simulink model "FMS1"  (R2018b)
settings: configuration reference "fms_config" (kept outside this file)
values from neighbouring files (symbols this model uses):
  FMS_EXPORT = Simulink.Parameter(FMS_EXPORT_VALUE)    [fms_model_init.m]
  FMS_PARAM = Simulink.Parameter(FMS_PARAM_VALUE)    [fms_model_init.m]
undefined symbols (not defined in the file or in its folder): actuator_cmd, ax_cmd, ay_cmd, az_cmd, cmd_mask, ControlMode, ctrl_mode, DiscIntNeverNeededParam, FMS_Cmd, FMS_CONST, home, mode, p_cmd, phi_cmd, PilotMode, psi_rate_cmd, q_cmd, r_cmd, reset, state, status, theta_cmd, throttle_cmd, timestamp, u_cmd, v_cmd, VehicleState, VehicleStatus, w_cmd, wp_consume, wp_current
libraries: simulink x119, FMT_Model_Lib x56, hdlsllib x13
(part 1 of 7)
settings Model: Creator=jc  LastModifiedBy=zouji
settings ConfigSetRef: SourceLocation=Base Workspace

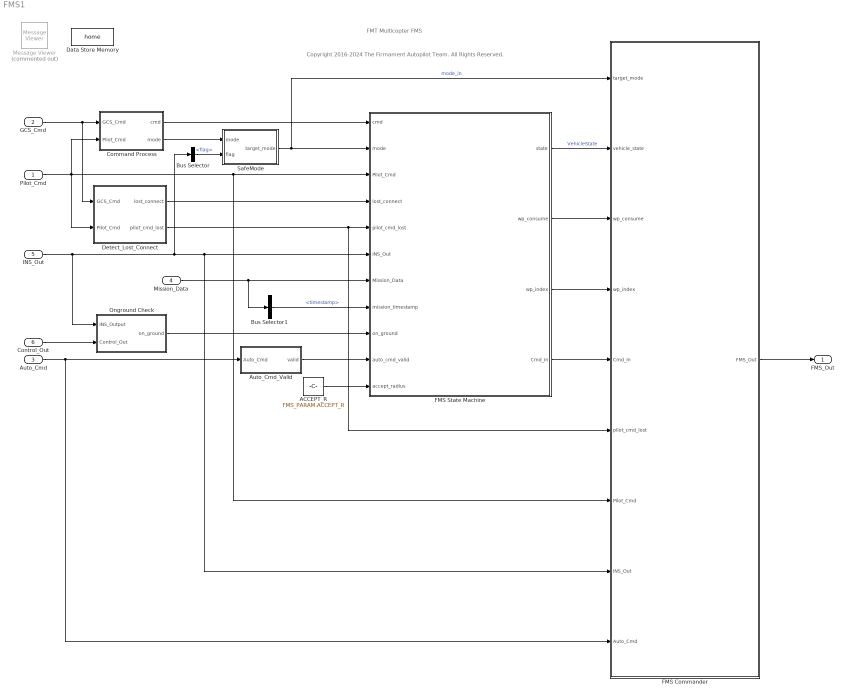
== system FMS1 ==
  note: Copyright 2016-2024 The Firmament Autopilot Team. All Rights Reserved.
  note: FMT Multicopter FMS
  Pilot_Cmd : Inport  OutDataTypeStr=Bus: Pilot_Cmd_Bus
  GCS_Cmd : Inport  Port=2  OutDataTypeStr=Bus: GCS_Cmd_Bus
  Auto_Cmd : Inport  Port=3  OutDataTypeStr=Bus: Auto_Cmd_Bus
  Mission_Data : Inport  Port=4  OutDataTypeStr=Bus: Mission_Data_Bus  BusOutputAsStruct=on
  INS_Out : Inport  Port=5  OutDataTypeStr=Bus: INS_Out_Bus
  Control_Out : Inport  Port=6  OutDataTypeStr=Bus: Control_Out_Bus
  ACCEPT_R : Constant  Value=FMS_PARAM.ACCEPT_R
  Auto_Cmd_Valid : Subsystem
  Bus Selector : BusSelector  OutputSignals=flag
  Bus Selector1 : BusSelector  OutputSignals=timestamp
  Command Process : Subsystem
  Data Store Memory : DataStoreMemory  DataStoreName=home  ReadBeforeWriteMsg=warning  WriteAfterWriteMsg=warning  WriteAfterReadMsg=warning  ShowAdditionalParam=off  OutDataTypeStr=single  Dimensions=4
  Detect_Lost_Connect : Subsystem
  FMS Commander : Subsystem  TreatAsAtomicUnit=on
  FMS State Machine : Stateflow chart  TreatAsAtomicUnit=on
  Message Viewer : MessageViewer  Commented=on  SavedRootId=#
  Onground Check : Subsystem
  SafeMode : Stateflow chart  TreatAsAtomicUnit=on
  FMS_Out : Outport  OutDataTypeStr=Bus: FMS_Out_Bus
  wires:
  Control_Out/1 -> Onground Check/2(Control_Out)
  Command Process/1(cmd) -> FMS State Machine/1(cmd)
  FMS State Machine/4(Cmd_In) -> FMS Commander/5(Cmd_In)
  Pilot_Cmd/1 -> Detect_Lost_Connect/2(Pilot_Cmd), FMS Commander/7(Pilot_Cmd), FMS State Machine/3(Pilot_Cmd), Command Process/2(Pilot_Cmd)
  INS_Out/1 -> Bus Selector/1, FMS Commander/8(INS_Out), FMS State Machine/6(INS_Out), Onground Check/1(INS_Output)
  Command Process/2(mode) -> SafeMode/1(mode)
  FMS Commander/1(FMS_Out) -> FMS_Out/1
  Onground Check/1(on_ground) -> FMS State Machine/9(on_ground)
  Bus Selector/1 -> SafeMode/2(flag)  "<flag>"
  GCS_Cmd/1 -> Command Process/1(GCS_Cmd), Detect_Lost_Connect/1(GCS_Cmd)
  SafeMode/1(target_mode) -> FMS Commander/1(target_mode), FMS State Machine/2(mode)  "mode_in"
  FMS State Machine/1(state) -> FMS Commander/2(vehicle_state)  "VehicleState"
  Mission_Data/1 -> Bus Selector1/1, FMS State Machine/7(Mission_Data)
  FMS State Machine/2(wp_consume) -> FMS Commander/3(wp_consume)
  Bus Selector1/1 -> FMS State Machine/8(mission_timestamp)  "<timestamp>"
  FMS State Machine/3(wp_index) -> FMS Commander/4(wp_index)
  ACCEPT_R/1 -> FMS State Machine/11(accept_radius)
  Auto_Cmd/1 -> FMS Commander/9(Auto_Cmd), Auto_Cmd_Valid/1(Auto_Cmd)
  Auto_Cmd_Valid/1(valid) -> FMS State Machine/10(auto_cmd_valid)
  Detect_Lost_Connect/1(lost_connect) -> FMS State Machine/4(lost_connect)
  Detect_Lost_Connect/2(pilot_cmd_lost) -> FMS Commander/6(pilot_cmd_lost), FMS State Machine/5(pilot_cmd_lost)

== system FMS1/Auto_Cmd_Valid ==
  Auto_Cmd : Inport
  Bus Selector1 : BusSelector  OutputSignals=frame
  Bus Selector2 : BusSelector  OutputSignals=timestamp
  Compare To Constant4 : simulink/Logic and Bit Operations/Compare To Constant  relop=<  const=1000  OutDataTypeStr=boolean
  Constant : Constant  Value=FMS_EXPORT.period  OutDataTypeStr=single
  Detect Change : simulink/Logic and Bit Operations/Detect Change  vinit=0  OutDataTypeStr=boolean
  Discrete-Time Integrator : DiscreteIntegrator  IntegratorMethod=Accumulation: Forward Euler  ExternalReset=sampled level  SampleTime=-1  OutDataTypeStr=uint32  SaturateOnIntegerOverflow=on  ICPrevOutput=DiscIntNeverNeededParam  ICPrevScaledInput=DiscIntNeverNeededParam
  Ever_Valid : Subsystem
  Interval Test : simulink/Logic and Bit Operations/Interval Test  IntervalClosedRight=on  uplimit=2  IntervalClosedLeft=on  lowlimit=0  OutDataTypeStr=boolean
  Logical Operator : Logic  Inputs=3  AllPortsSameDT=off  OutDataTypeStr=boolean
  valid : Outport
  wires:
  Constant/1 -> Discrete-Time Integrator/1
  Detect Change/1 -> Ever_Valid/1(in), Discrete-Time Integrator/2
  Discrete-Time Integrator/1 -> Compare To Constant4/1
  Auto_Cmd/1 -> Bus Selector1/1, Bus Selector2/1
  Compare To Constant4/1 -> Logical Operator/1
  Ever_Valid/1(out) -> Logical Operator/2
  Logical Operator/1 -> valid/1
  Bus Selector2/1 -> Detect Change/1  "<timestamp>"
  Bus Selector1/1 -> Interval Test/1  "<frame>"
  Interval Test/1 -> Logical Operator/3

== system FMS1/Command Process ==
  GCS_Cmd : Inport
  Pilot_Cmd : Inport  Port=2
  Check Valid : Subsystem
  Command PreProcess : Subsystem
  Mode PreProcess : Subsystem
  cmd : Outport
  mode : Outport  Port=2
  wires:
  GCS_Cmd/1 -> Mode PreProcess/2(GCS_Cmd), Command PreProcess/1(gcs_cmd)
  Pilot_Cmd/1 -> Command PreProcess/2(pilot_cmd), Check Valid/1(Pilot_Cmd), Mode PreProcess/3(Pilot_Cmd)
  Command PreProcess/1(cmd) -> cmd/1  "fms_cmd"
  Check Valid/1(pilot_cmd_valid) -> Mode PreProcess/1(pilot_cmd_valid)
  Mode PreProcess/1(mode) -> mode/1  "fms_mode"

== system FMS1/Detect_Lost_Connect ==
  GCS_Cmd : Inport
  Pilot_Cmd : Inport  Port=2
  Bus Selector : BusSelector  OutputSignals=timestamp
  Bus Selector1 : BusSelector  OutputSignals=timestamp
  Constant : Constant  Value=FMS_CONST.dt  OutDataTypeStr=single
  Constant1 : Constant  Value=FMS_PARAM.LOST_RETURN_EN
  Detect Change : simulink/Logic and Bit Operations/Detect Change  vinit=0  OutDataTypeStr=boolean
  Detect Change1 : simulink/Logic and Bit Operations/Detect Change  vinit=0  OutDataTypeStr=boolean
  Discrete-Time Integrator : DiscreteIntegrator  IntegratorMethod=Accumulation: Forward Euler  ExternalReset=sampled level  SampleTime=-1  OutDataTypeStr=single  SaturateOnIntegerOverflow=on  LimitOutput=on  UpperSaturationLimit=65535  LowerSaturationLimit=0  ICPrevOutput=DiscIntNeverNeededParam  ICPrevScaledInput=DiscIntNeverNeededParam
  Discrete-Time Integrator1 : DiscreteIntegrator  IntegratorMethod=Accumulation: Forward Euler  ExternalReset=sampled level  SampleTime=-1  OutDataTypeStr=single  SaturateOnIntegerOverflow=on  LimitOutput=on  UpperSaturationLimit=65535  LowerSaturationLimit=0  ICPrevOutput=DiscIntNeverNeededParam  ICPrevScaledInput=DiscIntNeverNeededParam
  Logical Operator : Logic  Operator=OR  Inputs=3  AllPortsSameDT=off  OutDataTypeStr=boolean
  Logical Operator1 : Logic  Operator=NOT  AllPortsSameDT=off  OutDataTypeStr=boolean
  Logical Operator2 : Logic  AllPortsSameDT=off  OutDataTypeStr=boolean
  timeout1_s : simulink/Logic and Bit Operations/Compare To Constant  relop=>=  const=FMS_PARAM.LOST_RETURN_TIME  OutDataTypeStr=boolean
  timeout2_s : simulink/Logic and Bit Operations/Compare To Constant  relop=>=  const=1  OutDataTypeStr=boolean
  lost_connect : Outport
  pilot_cmd_lost : Outport  Port=2
  wires:
  Constant/1 -> Discrete-Time Integrator1/1, Discrete-Time Integrator/1
  Discrete-Time Integrator/1 -> timeout1_s/1
  GCS_Cmd/1 -> Bus Selector/1
  Pilot_Cmd/1 -> Bus Selector1/1
  Bus Selector/1 -> Detect Change/1  "<timestamp>"
  Bus Selector1/1 -> Detect Change1/1  "<timestamp>"
  Detect Change/1 -> Logical Operator/1
  Detect Change1/1 -> Discrete-Time Integrator1/2, Logical Operator/2
  Constant1/1 -> Logical Operator2/2, Logical Operator1/1
  Logical Operator1/1 -> Logical Operator/3
  Logical Operator/1 -> Discrete-Time Integrator/2
  Logical Operator2/1 -> lost_connect/1
  timeout1_s/1 -> Logical Operator2/1
  Discrete-Time Integrator1/1 -> timeout2_s/1
  timeout2_s/1 -> pilot_cmd_lost/1

== system FMS1/FMS Commander ==
  target_mode : Inport
  vehicle_state : Inport  Port=2
  wp_consume : Inport  Port=3
  wp_index : Inport  Port=4
  Cmd_In : Inport  Port=5
  pilot_cmd_lost : Inport  Port=6
  Pilot_Cmd : Inport  Port=7
  INS_Out : Inport  Port=8
  Auto_Cmd : Inport  Port=9
  Commander : Subsystem
  FMS_Input : Subsystem  TreatAsAtomicUnit=on
  FMS_Out : Outport
  wires:
  target_mode/1 -> Commander/1(target_mode)
  FMS_Input/1(FMS_In) -> Commander/2(FMS_In)  "FMS_In"
  Commander/1(FMS_Out) -> FMS_Out/1
  vehicle_state/1 -> FMS_Input/1(state)
  wp_consume/1 -> FMS_Input/2(wp_consume)
  wp_index/1 -> FMS_Input/3(wp_index)
  Cmd_In/1 -> FMS_Input/4(Cmd_In)
  Pilot_Cmd/1 -> FMS_Input/6(Pilot_Cmd)
  INS_Out/1 -> FMS_Input/7(INS_Out)
  Auto_Cmd/1 -> FMS_Input/8(Auto_Cmd)
  pilot_cmd_lost/1 -> FMS_Input/5(pilot_cmd_lost)

== system FMS1/FMS State Machine/Vehicle.Arm.Auto.Mission.LLA2FLAT ==
  lla : Inport  OutDataTypeStr=double  PortDimensions=[1 3]
  llo : Inport  Port=2  OutDataTypeStr=double  Unit=deg  PortDimensions=[1 2]
  href : Inport  Port=3  OutDataTypeStr=double  Unit=m  PortDimensions=1
  psio : Inport  Port=4  OutDataTypeStr=double  Unit=deg  PortDimensions=1
  f : TriggerPort  TriggerType=function-call  VariantControl=(inherit)
      settings: CopyFcn=Stateflow.SLINSF.SimulinkMan.removeBlockPreDeleteFcn  PreDeleteFcn=Stateflow.SLINSF.SimulinkMan.unsafePredeleteFcn
  Data Type Conversion : DataTypeConversion  OutDataTypeStr=single
  LLA2FLAT : FMT_Model_Lib/Transformation/LLA2FLAT
      settings: SourceProductName=FMT Toolbox
  Signal Conversion : SignalConversion  OverrideOpt=off
  pos : Outport
  wires:
  LLA2FLAT/1 -> Signal Conversion/1
  lla/1 -> LLA2FLAT/1
  llo/1 -> LLA2FLAT/2
  href/1 -> LLA2FLAT/3
  psio/1 -> LLA2FLAT/4
  Signal Conversion/1 -> Data Type Conversion/1
  Data Type Conversion/1 -> pos/1

== system FMS1/FMS State Machine/Vehicle.PrepTakeoff ==
  xy_R : Inport  OutDataTypeStr=single  PortDimensions=2
  f : TriggerPort  TriggerType=function-call  VariantControl=(inherit)  StatesWhenEnabling=reset
      settings: CopyFcn=Stateflow.SLINSF.SimulinkMan.removeBlockPreDeleteFcn  PreDeleteFcn=Stateflow.SLINSF.SimulinkMan.unsafePredeleteFcn
  Constant : Constant  Value=FMS_PARAM.TAKEOFF_H
  Mux : Mux  Inputs=2
  Reshape : Reshape  OutputDimensionality=Column vector (2-D)
  sp_takeoff : Outport
  wires:
  Reshape/1 -> sp_takeoff/1
  xy_R/1 -> Mux/1
  Mux/1 -> Reshape/1
  Constant/1 -> Mux/2

== system FMS1/FMS State Machine/Vehicle.StickMoved ==
  stick_val : Inport  OutDataTypeStr=double  PortDimensions=4
  pilot_cmd : Inport  Port=2  OutDataTypeStr=Bus: Pilot_Cmd_Bus  PortDimensions=1
  f : TriggerPort  TriggerType=function-call  VariantControl=(inherit)
      settings: CopyFcn=Stateflow.SLINSF.SimulinkMan.removeBlockPreDeleteFcn  PreDeleteFcn=Stateflow.SLINSF.SimulinkMan.unsafePredeleteFcn
  Abs : Abs
  Bus Selector : BusSelector  OutputSignals=stick_yaw,stick_throttle,stick_roll,stick_pitch
  Compare To Constant : simulink/Logic and Bit Operations/Compare To Constant  relop=>=  const=0.1  OutDataTypeStr=boolean
  Max : MinMax  Function=max
  Mux : Mux
  Sum : Sum  Inputs=|+-
  moved : Outport
  wires:
  pilot_cmd/1 -> Bus Selector/1
  Bus Selector/1 -> Mux/1  "<stick_yaw>"
  Bus Selector/2 -> Mux/2  "<stick_throttle>"
  Bus Selector/3 -> Mux/3  "<stick_roll>"
  Bus Selector/4 -> Mux/4  "<stick_pitch>"
  stick_val/1 -> Sum/1
  Mux/1 -> Sum/2
  Sum/1 -> Abs/1
  Abs/1 -> Max/1
  Max/1 -> Compare To Constant/1
  Compare To Constant/1 -> moved/1

== system FMS1/Onground Check ==
  INS_Output : Inport
  Control_Out : Inport  Port=2
  Bus Selector : BusSelector  OutputSignals=quat
  Bus Selector1 : BusSelector  OutputSignals=actuator_cmd
  Bus Selector2 : BusSelector  OutputSignals=phi,theta
  Bus Selector3 : BusSelector  OutputSignals=ax,ay,az
  Constant : Constant  Value=4  OutDataTypeStr=uint16
  Cos : Trigonometry  Operator=cos
  Cos1 : Trigonometry  Operator=cos
  Divide : Product  Inputs=*/
  Divide1 : Product  Inputs=/*
  First Order LPF : FMT_Model_Lib/Filter/First Order LPF  fc=1/(2*pi*0.5)
      settings: SourceProductName=FMT Toolbox
  First Order LPF1 : FMT_Model_Lib/Filter/First Order LPF  fc=1/(2*pi*0.1)
      settings: SourceProductName=FMT Toolbox
  First Order LPF2 : FMT_Model_Lib/Filter/First Order LPF  fc=1/(2*pi*0.1)
      settings: SourceProductName=FMT Toolbox
  Interval Test : simulink/Logic and Bit Operations/Interval Test  IntervalClosedRight=on  uplimit=[0.5, 0.5, -9.806+0.5]  IntervalClosedLeft=on  lowlimit=[-0.5, -0.5, -9.806-0.5]  OutDataTypeStr=boolean
  Land_Lock_Thro : Constant  Value=FMS_PARAM.LAND_LOCK_THRO
  Logical Operator : Logic  Inputs=1  AllPortsSameDT=off  OutDataTypeStr=boolean
  Logical Operator1 : Logic  AllPortsSameDT=off  OutDataTypeStr=boolean
  Matrix Concatenate3 : Concatenate  NumInputs=3  ConcatenateDimension=2
  Multiply : Product  Multiplication=Matrix(*)
  Multiply1 : Product
  Quaternion To DCM : FMT_Model_Lib/Quaternion/Quaternion To DCM
      settings: SourceProductName=FMT Toolbox
  Relational Operator : RelationalOperator  Operator=<  OutDataTypeStr=boolean  RndMeth=Simplest
  Saturation : Saturate  UpperLimit=1  LowerLimit=0.9
  Selector : Selector  InputPortWidth=16  IndexOptions=Index vector (dialog)  Indices=[1:4]  OutputSizes=1
  Sum of Elements : Sum  Inputs=+
  Transpose : Math  Operator=transpose  SaturateOnIntegerOverflow=on
  on_ground : Outport
  wires:
  Bus Selector3/2 -> Matrix Concatenate3/2  "<ay>"
  Relational Operator/1 -> Logical Operator1/2
  Bus Selector3/3 -> Matrix Concatenate3/3  "<az>"
  Bus Selector1/1 -> Selector/1  "<actuator_cmd>"
  Bus Selector3/1 -> Matrix Concatenate3/1  "<ax>"
  Selector/1 -> Sum of Elements/1
  INS_Output/1 -> Bus Selector2/1, Bus Selector3/1, Bus Selector/1
  Control_Out/1 -> Bus Selector1/1
  Interval Test/1 -> Logical Operator/1
  Sum of Elements/1 -> Divide/1
  Constant/1 -> Divide/2
  First Order LPF/1 -> Interval Test/1
  Divide/1 -> First Order LPF2/1
  First Order LPF2/1 -> Relational Operator/1
  Logical Operator/1 -> Logical Operator1/1
  Logical Operator1/1 -> on_ground/1  "on_ground"
  Bus Selector/1 -> Quaternion To DCM/1  "<quat>"
  Quaternion To DCM/1 -> Transpose/1
  Matrix Concatenate3/1 -> Multiply/2
  Transpose/1 -> Multiply/1
  Multiply/1 -> First Order LPF/1
  Bus Selector2/1 -> Cos/1  "<phi>"
  Bus Selector2/2 -> Cos1/1  "<theta>"
  Cos/1 -> Multiply1/1
  Cos1/1 -> Multiply1/2
  Multiply1/1 -> Saturation/1
  Saturation/1 -> Divide1/1
  Divide1/1 -> First Order LPF1/1
  First Order LPF1/1 -> Relational Operator/2
  Land_Lock_Thro/1 -> Divide1/2

== system FMS1/Auto_Cmd_Valid/Ever_Valid ==
  in : Inport
  Constant1 : Constant  OutDataTypeStr=uint8
  Delay : Delay  DelayLength=1
  Switch : Switch  Criteria=u2 > Threshold
  out : Outport
  wires:
  Constant1/1 -> Switch/1
  Delay/1 -> Switch/3
  in/1 -> Switch/2
  Switch/1 -> out/1, Delay/1

== system FMS1/Command Process/Check Valid ==
  Pilot_Cmd : Inport
  Bus Selector1 : BusSelector  OutputSignals=timestamp
  Compare To Constant1 : simulink/Logic and Bit Operations/Compare To Constant  relop=<  const=500  OutDataTypeStr=boolean
  Constant1 : Constant  Value=FMS_EXPORT.period  OutDataTypeStr=single
  Detect Change1 : simulink/Logic and Bit Operations/Detect Change  vinit=0  OutDataTypeStr=boolean
  Discrete-Time Integrator1 : DiscreteIntegrator  IntegratorMethod=Accumulation: Forward Euler  ExternalReset=sampled level  SampleTime=-1  OutDataTypeStr=uint32  SaturateOnIntegerOverflow=on  ICPrevOutput=DiscIntNeverNeededParam  ICPrevScaledInput=DiscIntNeverNeededParam
  pilot_cmd_valid : Outport
  wires:
  Pilot_Cmd/1 -> Bus Selector1/1
  Compare To Constant1/1 -> pilot_cmd_valid/1
  Bus Selector1/1 -> Detect Change1/1  "<timestamp>"
  Constant1/1 -> Discrete-Time Integrator1/1
  Detect Change1/1 -> Discrete-Time Integrator1/2
  Discrete-Time Integrator1/1 -> Compare To Constant1/1

== system FMS1/Command Process/Command PreProcess ==
  gcs_cmd : Inport
  pilot_cmd : Inport  Port=2
  Bus Selector : BusSelector  OutputSignals=cmd_1
  Bus Selector1 : BusSelector  OutputSignals=cmd_1
  Bus Selector2 : BusSelector  OutputSignals=param
  Compare To Constant : simulink/Logic and Bit Operations/Compare To Constant  relop===  const=FMS_Cmd.SetHome  OutDataTypeStr=boolean
  Constant1 : Constant  Value=FMS_Cmd.None
  Data Type Conversion1 : DataTypeConversion  OutDataTypeStr=Enum: FMS_Cmd
  Data Type Conversion2 : DataTypeConversion  OutDataTypeStr=Enum: FMS_Cmd
  Detect Change3 : simulink/Logic and Bit Operations/Detect Change  vinit=0  OutDataTypeStr=boolean
  Detect Change4 : simulink/Logic and Bit Operations/Detect Change  vinit=0  OutDataTypeStr=boolean
  Selector : Selector  InputPortWidth=7  IndexOptions=Index vector (dialog)  Indices=[1:4]  OutputSizes=1
  SetHome : Subsystem  TreatAsAtomicUnit=on
  Switch1 : Switch  Criteria=u2 > Threshold
  Switch2 : Switch  Criteria=u2 > Threshold
  cmd : Outport
  wires:
  Bus Selector/1 -> Data Type Conversion1/1, Detect Change4/1  "<cmd_1>"
  pilot_cmd/1 -> Bus Selector1/1
  Switch1/1 -> cmd/1
  gcs_cmd/1 -> Bus Selector2/1, Bus Selector/1
  Bus Selector1/1 -> Data Type Conversion2/1, Detect Change3/1  "<cmd_1>"
  Detect Change3/1 -> Switch1/2
  Switch2/1 -> Switch1/3
  Detect Change4/1 -> Switch2/2
  Data Type Conversion2/1 -> Switch1/1
  Data Type Conversion1/1 -> Compare To Constant/1, Switch2/1
  Constant1/1 -> Switch2/3
  Compare To Constant/1 -> SetHome/Trigger
  Bus Selector2/1 -> Selector/1  "<param>"
  Selector/1 -> SetHome/1(home)

== system FMS1/Command Process/Mode PreProcess ==
  pilot_cmd_valid : Inport
  GCS_Cmd : Inport  Port=2
  Pilot_Cmd : Inport  Port=3
  Bus Selector1 : BusSelector  OutputSignals=mode
  Bus Selector2 : BusSelector  OutputSignals=mode
  Compare To Zero : simulink/Logic and Bit Operations/Compare To Zero  relop=~=  OutDataTypeStr=boolean
  Compare To Zero1 : simulink/Logic and Bit Operations/Compare To Zero  relop=~=  OutDataTypeStr=boolean
  Data Type Conversion1 : DataTypeConversion  OutDataTypeStr=Enum: PilotMode
  Data Type Conversion2 : DataTypeConversion  OutDataTypeStr=Enum: PilotMode
  Delay : Delay  DelayLength=1  InitialCondition=PilotMode.None
  Detect Change : simulink/Logic and Bit Operations/Detect Change  vinit=0  OutDataTypeStr=boolean
  Logical Operator : Logic  AllPortsSameDT=off  OutDataTypeStr=boolean
  Logical Operator1 : Logic  AllPortsSameDT=off  OutDataTypeStr=boolean
  Switch : Switch  Criteria=u2 > Threshold
  Switch1 : Switch  Criteria=u2 > Threshold
  mode : Outport
  wires:
  Bus Selector2/1 -> Compare To Zero/1, Detect Change/1, Data Type Conversion1/1  "<mode>"
  GCS_Cmd/1 -> Bus Selector2/1
  Pilot_Cmd/1 -> Bus Selector1/1
  Bus Selector1/1 -> Compare To Zero1/1, Data Type Conversion2/1  "<mode>"
  Logical Operator1/1 -> Switch/2
  Data Type Conversion2/1 -> Switch/1
  Switch/1 -> mode/1, Delay/1
  Delay/1 -> Switch1/3
  Compare To Zero/1 -> Logical Operator/2
  Data Type Conversion1/1 -> Switch1/1
  Switch1/1 -> Switch/3
  Detect Change/1 -> Logical Operator/1
  Logical Operator/1 -> Switch1/2
  pilot_cmd_valid/1 -> Logical Operator1/2
  Compare To Zero1/1 -> Logical Operator1/1

== system FMS1/FMS Commander/Commander ==
  target_mode : Inport
  FMS_In : Inport  Port=2
  Arm : Subsystem  TreatAsAtomicUnit=on
  Bus Selector1 : BusSelector  OutputSignals=vehicle_state
  Bus_Constructor : Subsystem
  Disarm : Subsystem  TreatAsAtomicUnit=on
  FMS_In1 : InportShadow  Port=2
  FMS_In2 : InportShadow  Port=2
  Merge : Merge  Inputs=3
  Standby : Subsystem  TreatAsAtomicUnit=on
  Switch Case : SwitchCase  CaseConditions={[VehicleState.Disarm,VehicleState.None], VehicleState.Standby}
  FMS_Out : Outport
  wires:
  Switch Case/3 -> Arm/Action
  Bus Selector1/1 -> Switch Case/1  "<vehicle_state>"
  FMS_In/1 -> Bus Selector1/1
  Standby/1(FMS_Out) -> Merge/2
  Arm/1(FMS_Out) -> Merge/3
  Switch Case/2 -> Standby/Action
  Switch Case/1 -> Disarm/Action
  Disarm/1(FMS_Out) -> Merge/1
  FMS_In1/1 -> Arm/1(FMS_In)
  Merge/1 -> Bus_Constructor/1(Bus_In)
  target_mode/1 -> Bus_Constructor/2(target_mode)
  FMS_In2/1 -> Bus_Constructor/3(FMS_In)
  Bus_Constructor/1(FMS_Out) -> FMS_Out/1

== system FMS1/FMS Commander/FMS_Input ==
  state : Inport
  wp_consume : Inport  Port=2
  wp_index : Inport  Port=3
  Cmd_In : Inport  Port=4
  pilot_cmd_lost : Inport  Port=5
  Pilot_Cmd : Inport  Port=6
  INS_Out : Inport  Port=7
  Auto_Cmd : Inport  Port=8
  Bus Creator : BusCreator  Inputs=8
  Signal Copy{,1..7} (8 alike) : SignalConversion  OverrideOpt=off
  FMS_In : Outport
  wires:
  Bus Creator/1 -> FMS_In/1
  Pilot_Cmd/1 -> Signal Copy2/1
  Auto_Cmd/1 -> Signal Copy/1
  INS_Out/1 -> Signal Copy1/1
  Signal Copy2/1 -> Bus Creator/6  "Pilot_Cmd"
  Signal Copy/1 -> Bus Creator/8  "Auto_Cmd"
  Signal Copy1/1 -> Bus Creator/7  "INS_Out"
  Cmd_In/1 -> Signal Copy3/1
  Signal Copy3/1 -> Bus Creator/4  "Cmd_In"
  wp_index/1 -> Signal Copy5/1
  Signal Copy5/1 -> Bus Creator/3  "wp_index"
  wp_consume/1 -> Signal Copy4/1
  Signal Copy4/1 -> Bus Creator/2  "wp_consume"
  state/1 -> Signal Copy6/1
  Signal Copy6/1 -> Bus Creator/1  "vehicle_state"
  pilot_cmd_lost/1 -> Signal Copy7/1
  Signal Copy7/1 -> Bus Creator/5  "pilot_cmd_lost"

== system FMS1/Command Process/Command PreProcess/SetHome ==
  home : Inport
  Trigger : TriggerPort  VariantControl=Variant
  Data Store Write : DataStoreWrite  DataStoreName=home
  wires:
  home/1 -> Data Store Write/1

== system FMS1/FMS Commander/Commander/Arm ==
  In Bus Element{,1..2,6..7} (5 alike) : Inport  PortName=FMS_In
  Action Port : ActionPort  InitializeStates=reset  ActionType=default
  Assist : Subsystem  TreatAsAtomicUnit=on
  Auto : Subsystem  TreatAsAtomicUnit=on
  Bus Selector : BusSelector  OutputSignals=vehicle_state
  Manual : Subsystem  TreatAsAtomicUnit=on
  Merge : Merge  Inputs=5
  SubMode : Subsystem  TreatAsAtomicUnit=on
  Switch Case : SwitchCase  CaseConditions={[VehicleState.Land,VehicleState.Return,VehicleState.Takeoff,VehicleState.Hold], [VehicleState.Offboard,VehicleState.Mission],[VehicleState.Acro,VehicleState.Stabilize,VehicleState.Altitude,VehicleState.Position],VehicleState.Manual}
  Unknown : Subsystem  TreatAsAtomicUnit=on
  FMS_Out : Outport
  wires:
  Merge/1 -> FMS_Out/1
  Switch Case/1 -> SubMode/Action
  Switch Case/2 -> Auto/Action
  Switch Case/3 -> Assist/Action
  Switch Case/4 -> Manual/Action
  SubMode/1(FMS_Out) -> Merge/1
  Auto/1(FMS_Out) -> Merge/2
  Assist/1(FMS_Out) -> Merge/3
  Manual/1(FMS_Out) -> Merge/4
  In Bus Element/1 -> SubMode/1(FMS_In)
  In Bus Element1/1 -> Assist/1(FMS_In)
  In Bus Element6/1 -> Auto/1(FMS_In)
  In Bus Element7/1 -> Manual/1(FMS_In)
  Switch Case/5 -> Unknown/Action
  Unknown/1(FMS_Out) -> Merge/5
  In Bus Element2/1 -> Bus Selector/1
  Bus Selector/1 -> Switch Case/1  "<vehicle_state>"

== system FMS1/FMS Commander/Commander/Bus_Constructor ==
  Bus_In : Inport
  target_mode : Inport  Port=2
  FMS_In : Inport  Port=3
  Bus Assignment : BusAssignment  AssignedSignals=timestamp,mode,wp_consume,wp_current,home
  Bus Selector : BusSelector  OutputSignals=wp_consume,wp_index
  Constant : Constant  OutDataTypeStr=uint8
  Data Store Read : DataStoreRead  DataStoreName=home
  Data Type Conversion : DataTypeConversion
  Sum : Sum  Inputs=-+|
  timestamp : Subsystem  mask{sample_time=FMS_EXPORT.period}
      mask prompts: sample_time "sample time (ms)"
  FMS_Out : Outport
  wires:
  Bus Selector/1 -> Bus Assignment/4  "<wp_consume>"
  target_mode/1 -> Data Type Conversion/1
  Bus_In/1 -> Bus Assignment/1
  Bus Assignment/1 -> FMS_Out/1
  Data Type Conversion/1 -> Bus Assignment/3
  FMS_In/1 -> Bus Selector/1
  timestamp/1(timestamp_ms) -> Bus Assignment/2
  Sum/1 -> Bus Assignment/5
  Data Store Read/1 -> Bus Assignment/6
  Bus Selector/2 -> Sum/2  "<wp_index>"
  Constant/1 -> Sum/1

== system FMS1/FMS Commander/Commander/Disarm ==
  Action Port : ActionPort  InitializeStates=reset  ActionType=case
  Bus Assignment : BusAssignment  AssignedSignals=reset,status,state
  Constant : Constant  Value=0  OutDataTypeStr=Bus: FMS_Out_Bus
  Constant1 : Constant  Value=VehicleStatus.Disarm
  Constant2 : Constant  OutDataTypeStr=Inherit: Inherit via back propagation
  Constant5 : Constant  Value=VehicleState.Disarm
  Data Type Conversion : DataTypeConversion
  Data Type Conversion1 : DataTypeConversion
  FMS_Out : Outport
  wires:
  Constant1/1 -> Data Type Conversion/1
  Constant2/1 -> Bus Assignment/2
  Bus Assignment/1 -> FMS_Out/1
  Constant/1 -> Bus Assignment/1
  Constant5/1 -> Data Type Conversion1/1
  Data Type Conversion/1 -> Bus Assignment/3
  Data Type Conversion1/1 -> Bus Assignment/4

== system FMS1/FMS Commander/Commander/Standby ==
  Action Port : ActionPort  InitializeStates=reset  ActionType=case
  Bus Assignment : BusAssignment  AssignedSignals=reset,status,state
  Constant : Constant  Value=0  OutDataTypeStr=Bus: FMS_Out_Bus
  Constant1 : Constant  Value=VehicleStatus.Standby
  Constant2 : Constant  OutDataTypeStr=Inherit: Inherit via back propagation
  Constant5 : Constant  Value=VehicleState.Standby
  Data Type Conversion1 : DataTypeConversion
  Data Type Conversion2 : DataTypeConversion
  FMS_Out : Outport
  wires:
  Constant/1 -> Bus Assignment/1
  Bus Assignment/1 -> FMS_Out/1
  Constant2/1 -> Bus Assignment/2
  Constant1/1 -> Data Type Conversion2/1
  Constant5/1 -> Data Type Conversion1/1
  Data Type Conversion2/1 -> Bus Assignment/3
  Data Type Conversion1/1 -> Bus Assignment/4

== system FMS1/FMS Commander/Commander/Arm/Assist ==
  In Bus Element{1..5} (5 alike) : Inport  PortName=FMS_In
  Action Port : ActionPort  InitializeStates=reset  ActionType=case
  Acro : Subsystem
      settings: UndoDeleteFcn=Stateflow.SLINSF.SimulinkMan.restorePreDeleteFcn  PreDeleteFcn=Stateflow.SLINSF.SimulinkMan.removePreDeleteFcn
  Altitude : Subsystem
      settings: UndoDeleteFcn=Stateflow.SLINSF.SimulinkMan.restorePreDeleteFcn  PreDeleteFcn=Stateflow.SLINSF.SimulinkMan.removePreDeleteFcn
  Bus Selector : BusSelector  OutputSignals=vehicle_state
  Merge : Merge  Inputs=5
  Position : Subsystem
      settings: UndoDeleteFcn=Stateflow.SLINSF.SimulinkMan.restorePreDeleteFcn  PreDeleteFcn=Stateflow.SLINSF.SimulinkMan.removePreDeleteFcn
  Stabilize : Subsystem
      settings: UndoDeleteFcn=Stateflow.SLINSF.SimulinkMan.restorePreDeleteFcn  PreDeleteFcn=Stateflow.SLINSF.SimulinkMan.removePreDeleteFcn
  Switch Case : SwitchCase  CaseConditions={VehicleState.Acro,VehicleState.Stabilize,VehicleState.Altitude,VehicleState.Position}
  Unknown : Subsystem  TreatAsAtomicUnit=on
  FMS_Out : Outport
  wires:
  In Bus Element1/1 -> Position/1(FMS_In)
  Switch Case/4 -> Position/Action
  Switch Case/3 -> Altitude/Action
  In Bus Element2/1 -> Altitude/1(FMS_In)
  Switch Case/2 -> Stabilize/Action
  In Bus Element3/1 -> Stabilize/1(FMS_In)
  In Bus Element4/1 -> Acro/1(FMS_In)
  Switch Case/1 -> Acro/Action
  Acro/1(FMS_Out) -> Merge/1
  Stabilize/1(FMS_Out) -> Merge/2
  Altitude/1(FMS_Out) -> Merge/3
  Position/1(FMS_Out) -> Merge/4
  Merge/1 -> FMS_Out/1
  Unknown/1(FMS_Out) -> Merge/5
  Switch Case/5 -> Unknown/Action
  In Bus Element5/1 -> Bus Selector/1
  Bus Selector/1 -> Switch Case/1  "<vehicle_state>"

== system FMS1/FMS Commander/Commander/Arm/Auto ==
  In Bus Element6 : Inport  PortName=FMS_In
  In Bus Element1 : Inport  PortName=FMS_In
  In Bus Element2 : Inport  PortName=FMS_In
  Action Port : ActionPort  InitializeStates=reset  ActionType=case
  Bus Selector : BusSelector  OutputSignals=vehicle_state
  Merge : Merge  Inputs=3
  Mission : Subsystem
      settings: UndoDeleteFcn=Stateflow.SLINSF.SimulinkMan.restorePreDeleteFcn  PreDeleteFcn=Stateflow.SLINSF.SimulinkMan.removePreDeleteFcn
  Offboard : Subsystem
      settings: UndoDeleteFcn=Stateflow.SLINSF.SimulinkMan.restorePreDeleteFcn  PreDeleteFcn=Stateflow.SLINSF.SimulinkMan.removePreDeleteFcn
  Switch Case : SwitchCase  CaseConditions={VehicleState.Offboard,VehicleState.Mission}
  Unknown : Subsystem  TreatAsAtomicUnit=on
  FMS_Out : Outport
  wires:
  Merge/1 -> FMS_Out/1
  In Bus Element6/1 -> Offboard/1(FMS_In)
  Switch Case/1 -> Offboard/Action
  In Bus Element1/1 -> Mission/1(FMS_In)
  Switch Case/2 -> Mission/Action
  Offboard/1(FMS_Out) -> Merge/1
  Mission/1(FMS_Out) -> Merge/2
  Unknown/1(FMS_Out) -> Merge/3
  Switch Case/3 -> Unknown/Action
  In Bus Element2/1 -> Bus Selector/1
  Bus Selector/1 -> Switch Case/1  "<vehicle_state>"

== system FMS1/FMS Commander/Commander/Arm/Manual ==
  In Bus Element7 : Inport  PortName=FMS_In
  Action Port : ActionPort  InitializeStates=reset  ActionType=case
  Bus Assignment : BusAssignment  AssignedSignals=reset,status,state
  Constant : Constant  Value=0  OutDataTypeStr=Bus: FMS_Out_Bus
  Constant1 : Constant  Value=VehicleStatus.Disarm
  Constant2 : Constant  OutDataTypeStr=Inherit: Inherit via back propagation
  Constant5 : Constant  Value=VehicleState.Manual
  Data Type Conversion : DataTypeConversion
  Data Type Conversion1 : DataTypeConversion
  Terminator : Terminator
  FMS_Out : Outport
  wires:
  Data Type Conversion1/1 -> Bus Assignment/4
  Data Type Conversion/1 -> Bus Assignment/3
  Constant5/1 -> Data Type Conversion1/1
  Constant/1 -> Bus Assignment/1
  Bus Assignment/1 -> FMS_Out/1
  Constant2/1 -> Bus Assignment/2
  Constant1/1 -> Data Type Conversion/1
  In Bus Element7/1 -> Terminator/1

== system FMS1/FMS Commander/Commander/Arm/SubMode ==
  In Bus Element{1..5} (5 alike) : Inport  PortName=FMS_In
  Action Port : ActionPort  InitializeStates=reset  ActionType=case
  Bus Selector : BusSelector  OutputSignals=vehicle_state
  Hold : Subsystem
      settings: UndoDeleteFcn=Stateflow.SLINSF.SimulinkMan.restorePreDeleteFcn  PreDeleteFcn=Stateflow.SLINSF.SimulinkMan.removePreDeleteFcn
  Land : Subsystem
      settings: UndoDeleteFcn=Stateflow.SLINSF.SimulinkMan.restorePreDeleteFcn  PreDeleteFcn=Stateflow.SLINSF.SimulinkMan.removePreDeleteFcn
  Merge : Merge  Inputs=5
  Return : Subsystem
      settings: UndoDeleteFcn=Stateflow.SLINSF.SimulinkMan.restorePreDeleteFcn  PreDeleteFcn=Stateflow.SLINSF.SimulinkMan.removePreDeleteFcn
  Switch Case : SwitchCase  CaseConditions={VehicleState.Takeoff, VehicleState.Land, VehicleState.Return,VehicleState.Hold}
  Takeoff : Subsystem
      settings: UndoDeleteFcn=Stateflow.SLINSF.SimulinkMan.restorePreDeleteFcn  PreDeleteFcn=Stateflow.SLINSF.SimulinkMan.removePreDeleteFcn
  Unknown : Subsystem  TreatAsAtomicUnit=on
  FMS_Out : Outport
  wires:
  Merge/1 -> FMS_Out/1
  In Bus Element1/1 -> Land/1(FMS_In)
  Land/1(FMS_Out) -> Merge/2
  Switch Case/2 -> Land/Action
  Switch Case/1 -> Takeoff/Action
  In Bus Element2/1 -> Takeoff/1(FMS_In)
  Takeoff/1(FMS_Out) -> Merge/1
  Switch Case/3 -> Return/Action
  In Bus Element3/1 -> Return/1(FMS_In)
  Return/1(FMS_Out) -> Merge/3
  Hold/1(FMS_Out) -> Merge/4
  In Bus Element4/1 -> Hold/1(FMS_In)
  Switch Case/4 -> Hold/Action
  Switch Case/5 -> Unknown/Action
  Unknown/1(FMS_Out) -> Merge/5
  In Bus Element5/1 -> Bus Selector/1
  Bus Selector/1 -> Switch Case/1  "<vehicle_state>"

== system FMS1/FMS Commander/Commander/Arm/Unknown ==
  Action Port : ActionPort  InitializeStates=reset  ActionType=default
  Bus Assignment : BusAssignment  AssignedSignals=reset,status,state,actuator_cmd
  Constant : Constant  Value=0  OutDataTypeStr=Bus: FMS_Out_Bus
  Constant1 : Constant  Value=VehicleStatus.Disarm
  Constant2 : Constant  OutDataTypeStr=Inherit: Inherit via back propagation
  Constant3 : Constant  Value=[1000;1000;1000;1000]  VectorParams1D=off  OutDataTypeStr=Inherit: Inherit via back propagation
  Constant4 : Constant  Value=zeros(12,1)  OutDataTypeStr=Inherit: Inherit via back propagation
  Constant5 : Constant  Value=VehicleState.Disarm
  Data Type Conversion : DataTypeConversion
  Data Type Conversion1 : DataTypeConversion
  Mux : Mux  Inputs=2
  FMS_Out : Outport
  wires:
  Mux/1 -> Bus Assignment/5
  Constant4/1 -> Mux/2
  Constant3/1 -> Mux/1
  Constant1/1 -> Data Type Conversion/1
  Constant2/1 -> Bus Assignment/2
  Bus Assignment/1 -> FMS_Out/1
  Constant/1 -> Bus Assignment/1
  Constant5/1 -> Data Type Conversion1/1
  Data Type Conversion/1 -> Bus Assignment/3
  Data Type Conversion1/1 -> Bus Assignment/4

== system FMS1/FMS Commander/Commander/Bus_Constructor/timestamp ==
  Constant : Constant  Value=sample_time
  Data Type Conversion : DataTypeConversion  OutDataTypeStr=uint32
  Discrete-Time Integrator : DiscreteIntegrator  IntegratorMethod=Accumulation: Forward Euler  SampleTime=-1  ICPrevOutput=DiscIntNeverNeededParam  ICPrevScaledInput=DiscIntNeverNeededParam
  timestamp_ms : Outport
  wires:
  Discrete-Time Integrator/1 -> Data Type Conversion/1
  Constant/1 -> Discrete-Time Integrator/1
  Data Type Conversion/1 -> timestamp_ms/1

== system FMS1/FMS Commander/Commander/Arm/Assist/Acro ==
  FMS_In : Inport
  Action Port : ActionPort  InitializeStates=reset  ActionType=case
      settings: CopyFcn=Stateflow.SLINSF.SimulinkMan.removeBlockPreDeleteFcn
  Angular Rate Command : Subsystem
  Bus Assignment : BusAssignment  AssignedSignals=status,state,ctrl_mode,p_cmd,q_cmd,r_cmd,throttle_cmd
  Constant : Constant  Value=0  OutDataTypeStr=Bus: FMS_Out_Bus
  Constant1 : Constant  Value=VehicleState.Acro
  Constant2 : Constant  Value=ControlMode.Acro
  Constant5 : Constant  Value=VehicleStatus.Arm
  Data Type Conversion : DataTypeConversion
  Data Type Conversion1 : DataTypeConversion
  Data Type Conversion2 : DataTypeConversion
  Throttle Command : Subsystem
  FMS_Out : Outport
  wires:
  Data Type Conversion2/1 -> Bus Assignment/4
  Constant2/1 -> Data Type Conversion2/1
  Data Type Conversion1/1 -> Bus Assignment/3
  Constant1/1 -> Data Type Conversion1/1
  Data Type Conversion/1 -> Bus Assignment/2
  Bus Assignment/1 -> FMS_Out/1
  Throttle Command/1(throttle_cmd) -> Bus Assignment/8
  Constant/1 -> Bus Assignment/1
  Constant5/1 -> Data Type Conversion/1
  Angular Rate Command/1(p_cmd_radPs) -> Bus Assignment/5
  Angular Rate Command/2(q_cmd_radPs) -> Bus Assignment/6
  Angular Rate Command/3(r_cmd_radPs) -> Bus Assignment/7
  FMS_In/1 -> Throttle Command/1(FMS_In), Angular Rate Command/1(FMS_In)

== system FMS1/FMS Commander/Commander/Arm/Assist/Altitude ==
  In Bus Element1 : Inport  PortName=FMS_In
  Action Port : ActionPort  InitializeStates=reset  ActionType=case
      settings: CopyFcn=Stateflow.SLINSF.SimulinkMan.removeBlockPreDeleteFcn
  Altitude Command : Subsystem
  Attitude Command : Subsystem
  Bus Assignment : BusAssignment  AssignedSignals=status,state,ctrl_mode,phi_cmd,theta_cmd,psi_rate_cmd,w_cmd
  Constant : Constant  Value=0  OutDataTypeStr=Bus: FMS_Out_Bus
  Constant1 : Constant  Value=VehicleState.Altitude
  Constant2 : Constant  Value=ControlMode.ALTCTL
  Constant5 : Constant  Value=VehicleStatus.Arm
  Data Type Conversion1 : DataTypeConversion
  Data Type Conversion2 : DataTypeConversion
  Data Type Conversion3 : DataTypeConversion
  Heading Command : Subsystem
  FMS_Out : Outport
  wires:
  Constant5/1 -> Data Type Conversion1/1
  Constant/1 -> Bus Assignment/1
  Heading Command/1(psi_rate_cmd_radPs) -> Bus Assignment/7
  Altitude Command/1(w_cmd_mPs) -> Bus Assignment/8
  Attitude Command/1(phi_cmd_radPs) -> Bus Assignment/5
  Attitude Command/2(theta_cmd_radPs) -> Bus Assignment/6
  Bus Assignment/1 -> FMS_Out/1
  Data Type Conversion1/1 -> Bus Assignment/2
  Constant1/1 -> Data Type Conversion2/1
  Data Type Conversion2/1 -> Bus Assignment/3
  Data Type Conversion3/1 -> Bus Assignment/4
  Constant2/1 -> Data Type Conversion3/1
  In Bus Element1/1 -> Attitude Command/1(FMS_In), Heading Command/1(FMS_In), Altitude Command/1(FMS_In)

== system FMS1/FMS Commander/Commander/Arm/Assist/Position ==
  FMS_In : Inport
  Action Port : ActionPort  InitializeStates=reset  ActionType=case
      settings: CopyFcn=Stateflow.SLINSF.SimulinkMan.removeBlockPreDeleteFcn
  Altitude Command : Subsystem
  Bus Assignment : BusAssignment  AssignedSignals=status,state,ctrl_mode,psi_rate_cmd,u_cmd,v_cmd,w_cmd
  Constant : Constant  Value=0  OutDataTypeStr=Bus: FMS_Out_Bus
  Constant1 : Constant  Value=VehicleState.Position
  Constant2 : Constant  Value=ControlMode.POSCTL
  Constant5 : Constant  Value=VehicleStatus.Arm
  Data Type Conversion : DataTypeConversion
  Data Type Conversion1 : DataTypeConversion
  Data Type Conversion2 : DataTypeConversion
  Heading Command : Subsystem
  Position Command : Subsystem
  FMS_Out : Outport
  wires:
  Bus Assignment/1 -> FMS_Out/1
  Altitude Command/1(w_cmd_mPs) -> Bus Assignment/8
  Constant/1 -> Bus Assignment/1
  Position Command/1(u_cmd_mPs) -> Bus Assignment/6
  Constant5/1 -> Data Type Conversion/1
  Position Command/2(v_cmd_mPs) -> Bus Assignment/7
  Heading Command/1(psi_rate_cmd_radPs) -> Bus Assignment/5
  Data Type Conversion/1 -> Bus Assignment/2
  Constant1/1 -> Data Type Conversion1/1
  Data Type Conversion1/1 -> Bus Assignment/3
  Constant2/1 -> Data Type Conversion2/1
  Data Type Conversion2/1 -> Bus Assignment/4
  FMS_In/1 -> Heading Command/1(FMS_In), Altitude Command/1(FMS_In), Position Command/1(FMS_In)

== system FMS1/FMS Commander/Commander/Arm/Assist/Stabilize ==
  FMS_In : Inport
  Action Port : ActionPort  InitializeStates=reset  ActionType=case
      settings: CopyFcn=Stateflow.SLINSF.SimulinkMan.removeBlockPreDeleteFcn
  Attitude Command : Subsystem
  Bus Assignment : BusAssignment  AssignedSignals=status,state,ctrl_mode,phi_cmd,theta_cmd,psi_rate_cmd,throttle_cmd
  Constant : Constant  Value=0  OutDataTypeStr=Bus: FMS_Out_Bus
  Constant1 : Constant  Value=VehicleState.Stabilize
  Constant2 : Constant  Value=ControlMode.Stabilize
  Constant5 : Constant  Value=VehicleStatus.Arm
  Data Type Conversion : DataTypeConversion
  Data Type Conversion1 : DataTypeConversion
  Data Type Conversion2 : DataTypeConversion
  Heading Command : Subsystem
  Throttle Command : Subsystem
  FMS_Out : Outport
  wires:
  Constant5/1 -> Data Type Conversion/1
  Heading Command/1(psi_rate_cmd_radPs) -> Bus Assignment/7
  Constant/1 -> Bus Assignment/1
  Attitude Command/1(phi_cmd_radPs) -> Bus Assignment/5
  Throttle Command/1(throttle_cmd) -> Bus Assignment/8
  Attitude Command/2(theta_cmd_radPs) -> Bus Assignment/6
  FMS_In/1 -> Attitude Command/1(FMS_In), Throttle Command/1(FMS_In), Heading Command/1(FMS_In)
  Bus Assignment/1 -> FMS_Out/1
  Data Type Conversion/1 -> Bus Assignment/2
  Constant1/1 -> Data Type Conversion1/1
  Data Type Conversion1/1 -> Bus Assignment/3
  Constant2/1 -> Data Type Conversion2/1
  Data Type Conversion2/1 -> Bus Assignment/4

== system FMS1/FMS Commander/Commander/Arm/Assist/Unknown ==
  Action Port : ActionPort  InitializeStates=reset  ActionType=default
  Bus Assignment : BusAssignment  AssignedSignals=reset,status,state,actuator_cmd
  Constant : Constant  Value=0  OutDataTypeStr=Bus: FMS_Out_Bus
  Constant1 : Constant  Value=VehicleStatus.Disarm
  Constant2 : Constant  OutDataTypeStr=Inherit: Inherit via back propagation
  Constant3 : Constant  Value=[1000;1000;1000;1000]  VectorParams1D=off  OutDataTypeStr=Inherit: Inherit via back propagation
  Constant4 : Constant  Value=zeros(12,1)  OutDataTypeStr=Inherit: Inherit via back propagation
  Constant5 : Constant  Value=VehicleState.Disarm
  Data Type Conversion : DataTypeConversion
  Data Type Conversion1 : DataTypeConversion
  Mux : Mux  Inputs=2
  FMS_Out : Outport
  wires:
  Mux/1 -> Bus Assignment/5
  Constant4/1 -> Mux/2
  Constant3/1 -> Mux/1
  Constant1/1 -> Data Type Conversion/1
  Constant2/1 -> Bus Assignment/2
  Bus Assignment/1 -> FMS_Out/1
  Constant/1 -> Bus Assignment/1
  Constant5/1 -> Data Type Conversion1/1
  Data Type Conversion/1 -> Bus Assignment/3
  Data Type Conversion1/1 -> Bus Assignment/4

== system FMS1/FMS Commander/Commander/Arm/Auto/Mission ==
  FMS_In : Inport
  Action Port : ActionPort  InitializeStates=reset  ActionType=case
      settings: CopyFcn=Stateflow.SLINSF.SimulinkMan.removeBlockPreDeleteFcn
  Bus Selector : BusSelector  OutputSignals=wp_index
  Detect Change : simulink/Logic and Bit Operations/Detect Change  vinit=0  OutDataTypeStr=boolean
  Mission_SubSystem : Subsystem  TreatAsAtomicUnit=on
  FMS_Out : Outport
  wires:
  Mission_SubSystem/1(FMS_Out) -> FMS_Out/1
  FMS_In/1 -> Bus Selector/1, Mission_SubSystem/1(FMS_In)
  Bus Selector/1 -> Detect Change/1  "<wp_index>"
  Detect Change/1 -> Mission_SubSystem/Reset

== system FMS1/FMS Commander/Commander/Arm/Auto/Offboard ==
  FMS_In : Inport
  Action Port : ActionPort  InitializeStates=reset  ActionType=case
      settings: CopyFcn=Stateflow.SLINSF.SimulinkMan.removeBlockPreDeleteFcn
  Acc_Command : Subsystem
  Bus Assignment : BusAssignment  AssignedSignals=status,state,ctrl_mode,p_cmd,q_cmd,r_cmd,phi_cmd,theta_cmd,throttle_cmd,ax_cmd,ay_cmd,az_cmd,psi_rate_cmd,u_cmd,v_cmd,w_cmd,cmd_mask
  Bus Selector : BusSelector  OutputSignals=Auto_Cmd.p_cmd,Auto_Cmd.q_cmd,Auto_Cmd.r_cmd,Auto_Cmd.phi_cmd,Auto_Cmd.theta_cmd,Auto_Cmd.throttle_cmd
  Command_Mask : Subsystem
  Constant : Constant  Value=0  OutDataTypeStr=Bus: FMS_Out_Bus
  Constant1 : Constant  Value=VehicleStatus.Arm
  Constant2 : Constant  Value=VehicleState.Offboard
  Constant3 : Constant  Value=ControlMode.Offboard
  Data Type Conversion : DataTypeConversion
  Data Type Conversion1 : DataTypeConversion
  Data Type Conversion2 : DataTypeConversion
  Heading_Command : Subsystem
  Velocity_Command : Subsystem
  FMS_Out : Outport
  wires:
  Bus Assignment/1 -> FMS_Out/1
  Constant/1 -> Bus Assignment/1
  Constant1/1 -> Data Type Conversion/1
  Data Type Conversion/1 -> Bus Assignment/2
  Constant2/1 -> Data Type Conversion1/1
  Data Type Conversion1/1 -> Bus Assignment/3
  Data Type Conversion2/1 -> Bus Assignment/4
  Constant3/1 -> Data Type Conversion2/1
  FMS_In/1 -> Command_Mask/1(FMS_In), Velocity_Command/1(FMS_In), Heading_Command/1(FMS_In), Acc_Command/1(FMS_In), Bus Selector/1
  Bus Selector/1 -> Bus Assignment/5  "<p_cmd>"
  Bus Selector/2 -> Bus Assignment/6  "<q_cmd>"
  Bus Selector/3 -> Bus Assignment/7  "<r_cmd>"
  Bus Selector/4 -> Bus Assignment/8  "<phi_cmd>"
  Bus Selector/5 -> Bus Assignment/9  "<theta_cmd>"
  Heading_Command/1(psi_rate_cmd) -> Bus Assignment/14
  Velocity_Command/1(u_cmd) -> Bus Assignment/15
  Velocity_Command/2(v_cmd) -> Bus Assignment/16
  Velocity_Command/3(w_cmd) -> Bus Assignment/17
  Command_Mask/1(cmd_mask) -> Bus Assignment/18
  Bus Selector/6 -> Bus Assignment/10  "<throttle_cmd>"
  Acc_Command/1(ax_cmd) -> Bus Assignment/11
  Acc_Command/2(ay_cmd) -> Bus Assignment/12
  Acc_Command/3(az_cmd) -> Bus Assignment/13

== system FMS1/FMS Commander/Commander/Arm/Auto/Unknown ==
  Action Port : ActionPort  InitializeStates=reset  ActionType=default
  Bus Assignment : BusAssignment  AssignedSignals=reset,status,state,actuator_cmd
  Constant : Constant  Value=0  OutDataTypeStr=Bus: FMS_Out_Bus
  Constant1 : Constant  Value=VehicleStatus.Disarm
  Constant2 : Constant  OutDataTypeStr=Inherit: Inherit via back propagation
  Constant3 : Constant  Value=[1000;1000;1000;1000]  VectorParams1D=off  OutDataTypeStr=Inherit: Inherit via back propagation
  Constant4 : Constant  Value=zeros(12,1)  OutDataTypeStr=Inherit: Inherit via back propagation
  Constant5 : Constant  Value=VehicleState.Disarm
  Data Type Conversion : DataTypeConversion
  Data Type Conversion1 : DataTypeConversion
  Mux : Mux  Inputs=2
  FMS_Out : Outport
  wires:
  Mux/1 -> Bus Assignment/5
  Constant4/1 -> Mux/2
  Constant3/1 -> Mux/1
  Constant1/1 -> Data Type Conversion/1
  Constant2/1 -> Bus Assignment/2
  Bus Assignment/1 -> FMS_Out/1
  Constant/1 -> Bus Assignment/1
  Constant5/1 -> Data Type Conversion1/1
  Data Type Conversion/1 -> Bus Assignment/3
  Data Type Conversion1/1 -> Bus Assignment/4

== system FMS1/FMS Commander/Commander/Arm/SubMode/Hold ==
  FMS_In : Inport
  Action Port : ActionPort  InitializeStates=reset  ActionType=case
      settings: CopyFcn=Stateflow.SLINSF.SimulinkMan.removeBlockPreDeleteFcn
  Altitude Hold : Subsystem
  Bus Assignment : BusAssignment  AssignedSignals=status,state,ctrl_mode,psi_rate_cmd,u_cmd,v_cmd,w_cmd
  Constant : Constant  Value=0  OutDataTypeStr=Bus: FMS_Out_Bus
  Constant1 : Constant  Value=VehicleState.Hold
  Constant2 : Constant  Value=ControlMode.POSCTL
  Constant5 : Constant  Value=VehicleStatus.Arm
  Data Type Conversion : DataTypeConversion
  Data Type Conversion1 : DataTypeConversion
  Data Type Conversion2 : DataTypeConversion
  Heading Hold : Subsystem
  Position Hold : Subsystem
  FMS_Out : Outport
  wires:
  Bus Assignment/1 -> FMS_Out/1
  Altitude Hold/1(w_cmd_mPs) -> Bus Assignment/8
  Constant/1 -> Bus Assignment/1
  Position Hold/1(u_cmd_mPs) -> Bus Assignment/6
  Constant5/1 -> Data Type Conversion/1
  Position Hold/2(v_cmd_mPs) -> Bus Assignment/7
  Heading Hold/1(psi_rate_cmd_radPs) -> Bus Assignment/5
  Data Type Conversion/1 -> Bus Assignment/2
  Constant1/1 -> Data Type Conversion1/1
  Data Type Conversion1/1 -> Bus Assignment/3
  Constant2/1 -> Data Type Conversion2/1
  Data Type Conversion2/1 -> Bus Assignment/4
  FMS_In/1 -> Heading Hold/1(FMS_In), Altitude Hold/1(FMS_In), Position Hold/1(FMS_In)

== system FMS1/FMS Commander/Commander/Arm/SubMode/Land ==
  FMS_In : Inport
  Action Port : ActionPort  InitializeStates=reset  ActionType=case
      settings: CopyFcn=Stateflow.SLINSF.SimulinkMan.removeBlockPreDeleteFcn
  Assist Land Speed : Subsystem
  Bus Assignment1 : BusAssignment  AssignedSignals=status,state,ctrl_mode,psi_rate_cmd,u_cmd,v_cmd,w_cmd
  Bus Selector : BusSelector  OutputSignals=Cmd_In.sp_waypoint
  Constant : Constant  Value=0  OutDataTypeStr=Inherit: Inherit via back propagation
  Constant1 : Constant  Value=0  OutDataTypeStr=Bus: FMS_Out_Bus
  Constant2 : Constant  Value=ControlMode.POSCTL
  Constant3 : Constant  Value=VehicleState.Land
  Constant6 : Constant  Value=VehicleStatus.Arm
  Data Type Conversion : DataTypeConversion
  Data Type Conversion1 : DataTypeConversion
  Data Type Conversion2 : DataTypeConversion
  Position Command : Subsystem
  Selector : Selector  InputPortWidth=3  IndexOptions=Index vector (dialog)  Indices=[1 2]  OutputSizes=1
  FMS_Out : Outport
  wires:
  Selector/1 -> Position Command/2(land_xy_R)
  Bus Assignment1/1 -> FMS_Out/1
  Constant1/1 -> Bus Assignment1/1
  Position Command/1(u_cmd_mPs) -> Bus Assignment1/6
  Position Command/2(v_cmd_mPs) -> Bus Assignment1/7
  Constant/1 -> Bus Assignment1/5
  Constant2/1 -> Data Type Conversion2/1
  Constant6/1 -> Data Type Conversion/1
  Data Type Conversion/1 -> Bus Assignment1/2
  Constant3/1 -> Data Type Conversion1/1
  Data Type Conversion1/1 -> Bus Assignment1/3
  Data Type Conversion2/1 -> Bus Assignment1/4
  Bus Selector/1 -> Selector/1  "<sp_waypoint>"
  FMS_In/1 -> Assist Land Speed/1(FMS_In), Position Command/1(FMS_In), Bus Selector/1
  Assist Land Speed/1(w_cmd_mPs) -> Bus Assignment1/8

== system FMS1/FMS Commander/Commander/Arm/SubMode/Return ==
  FMS_In : Inport
  Action Port : ActionPort  InitializeStates=reset  ActionType=case
      settings: CopyFcn=Stateflow.SLINSF.SimulinkMan.removeBlockPreDeleteFcn
  Bus Assignment1 : BusAssignment  AssignedSignals=status,state,ctrl_mode,u_cmd,v_cmd,w_cmd,psi_rate_cmd
  Constant1 : Constant  Value=VehicleState.Return
  Constant2 : Constant  Value=0  OutDataTypeStr=Bus: FMS_Out_Bus
  Constant3 : Constant  Value=ControlMode.POSCTL
  Constant6 : Constant  Value=VehicleStatus.Arm
  Data Type Conversion : DataTypeConversion
  Data Type Conversion1 : DataTypeConversion
  Data Type Conversion2 : DataTypeConversion
  Heading Commander : Subsystem
  L1 : Constant  Value=FMS_PARAM.L1  OutDataTypeStr=single
  Sum : Sum  Inputs=+-|
  Velocity Commander1 : Subsystem
  Way Points : Subsystem
  FMS_Out : Outport
  wires:
  Sum/1 -> Heading Commander/2(p1p2)
  Way Points/2(p2) -> Velocity Commander1/2(p2), Sum/1
  Way Points/3(p3) -> Velocity Commander1/3(p3)
  L1/1 -> Velocity Commander1/4(L1)
  Constant3/1 -> Data Type Conversion2/1
  Way Points/1(p1) -> Velocity Commander1/1(p1), Sum/2
  Constant2/1 -> Bus Assignment1/1
  Heading Commander/2(psi_rad_cmd) -> Bus Assignment1/8
  Bus Assignment1/1 -> FMS_Out/1
  Data Type Conversion/1 -> Bus Assignment1/2
  Constant6/1 -> Data Type Conversion/1
  Data Type Conversion1/1 -> Bus Assignment1/3
  Data Type Conversion2/1 -> Bus Assignment1/4
  Constant1/1 -> Data Type Conversion1/1
  FMS_In/1 -> Velocity Commander1/5(FMS_In), Heading Commander/1(FMS_In), Way Points/1(FMS_In)
  Velocity Commander1/1(u_cmd) -> Bus Assignment1/5
  Velocity Commander1/2(v_cmd) -> Bus Assignment1/6
  Velocity Commander1/3(w_cmd) -> Bus Assignment1/7
  Heading Commander/1(psi_err_rad) -> Velocity Commander1/6(psi_err_rad)
